simulink model "hqd_clarke"  (R2022b)
settings: Solver=FixedStepAuto  StartTime=0.0  StopTime=1.0  RelTol=1e-3
libraries: simulink x1
settings Model: Creator=15403  LastModifiedBy=15403
settings OptimizationCC: DefaultParameterBehavior=Inlined  UseDivisionForNetSlopeComputation=on  GainParamInheritBuiltInType=on  UseFloatMulNetSlope=on  InlineInvariantSignals=on  PassReuseOutputArgsAs=Individual arguments  ZeroExternalMemoryAtStartup=off  ZeroInternalMemoryAtStartup=off  NoFixptDivByZeroProtection=on  EfficientFloat2IntCast=on  LifeSpan=1  OptimizeBlockOrder=speed  DifferentSizesBufferReuse=on  EfficientTunableParamExpr=on
settings DebuggingCC: ParameterPrecisionLossMsg=none  ParameterTunabilityLossMsg=error
settings HardwareCC: ProdBitPerPointer=32  ProdBitPerSizeT=32  ProdBitPerPtrDiffT=32  ProdLargestAtomicInteger=Long  ProdLargestAtomicFloat=Double  ProdWordSize=32  ProdLongLongMode=on  ProdHWDeviceType=ARM Compatible->ARM Cortex-M
settings SFSimCC: MATLABDynamicMemAlloc=off
settings RTWCC: Description=Embedded Coder  SystemTargetFile=ert.tlc  TemplateMakefile=ert_default_tmf
settings CodeAppCC: ForceParamTrailComments=on  IgnoreCustomStorageClasses=off  OperatorAnnotations=on  SimulinkDataObjDesc=on  SFDataObjDesc=on  CustomSymbolStrGlobalVar=rt$N$M  CustomSymbolStrType=$N$M  CustomSymbolStrFcn=$N$M$F  CustomSymbolStrMacro=$N$M  InsertBlockDesc=on
settings ERTTargetCC: TargetLangStandard=C99 (ISO)  GenerateSampleERTMain=on  IncludeMdlTerminateFcn=off  CombineSignalStateStructs=on  SupportComplex=off  SupportContinuousTime=on  SupportNonInlinedSFcns=on  InlinedParameterPlacement=NonHierarchical  ERTCustomFileTemplate=example_file_process.tlc  ERTFilePackagingFormat=CompactWithDataFile

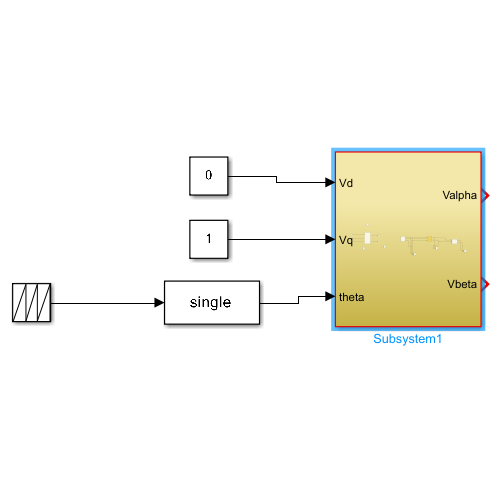
[thumbnail: Simulink's stored preview of the top-level diagram]
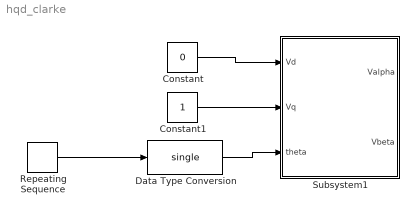
== system hqd_clarke ==
  Constant : Constant  Value=0  OutDataTypeStr=single
  Constant1 : Constant  OutDataTypeStr=single
  Data Type Conversion : DataTypeConversion  OutDataTypeStr=single  SaturateOnIntegerOverflow=off  RndMeth=Floor
  Repeating Sequence : simulink/Sources/Repeating Sequence  rep_seq_t=[0 0.1]  rep_seq_y=[0 2 * pi]
  Subsystem1 : Subsystem
  wires:
  Repeating Sequence/1 -> Data Type Conversion/1
  Constant/1 -> Subsystem1/1(Vd)
  Constant1/1 -> Subsystem1/2(Vq)
  Data Type Conversion/1 -> Subsystem1/3(theta)

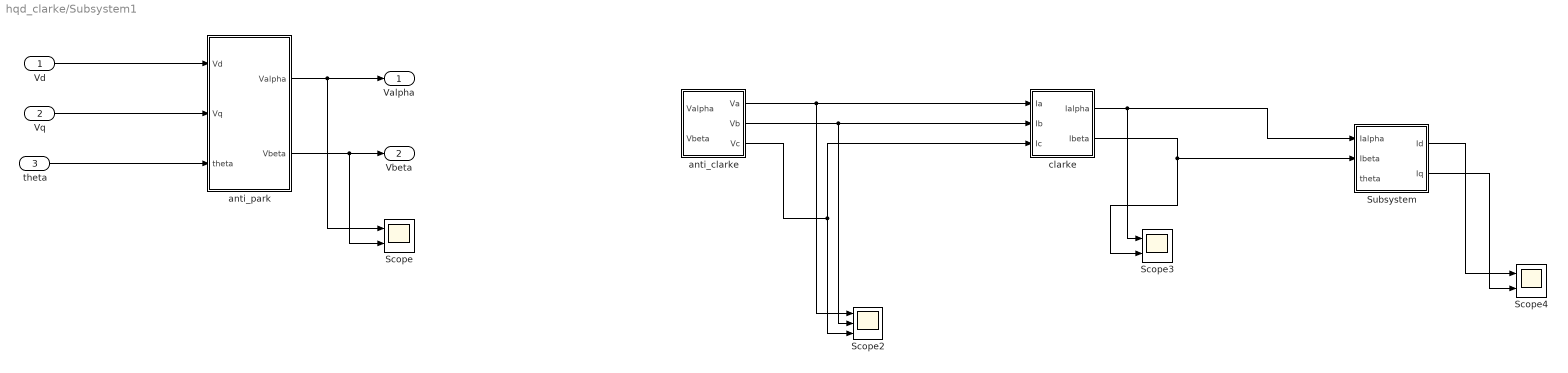
== system hqd_clarke/Subsystem1 ==
  Vd : Inport
  Vq : Inport  Port=2
  theta : Inport  Port=3
  Scope : Scope  NumInputPorts=2
  Scope2 : Scope  NumInputPorts=3
  Scope3 : Scope  NumInputPorts=2
  Scope4 : Scope  NumInputPorts=2
  Subsystem : Subsystem
  anti_clarke : Subsystem
  anti_park : Subsystem
  clarke : Subsystem
  Valpha : Outport
  Vbeta : Outport  Port=2
  wires:
  clarke/2(Ibeta) -> Scope3/2, Subsystem/2(Ibeta)
  anti_clarke/1(Va) -> clarke/1(Ia), Scope2/1
  Subsystem/1(Id) -> Scope4/1
  Subsystem/2(Iq) -> Scope4/2
  anti_clarke/3(Vc) -> clarke/3(Ic), Scope2/3
  anti_clarke/2(Vb) -> clarke/2(Ib), Scope2/2
  clarke/1(Ialpha) -> Subsystem/1(Ialpha), Scope3/1
  Vd/1 -> anti_park/1(Vd)
  Vq/1 -> anti_park/2(Vq)
  theta/1 -> anti_park/3(theta)
  anti_park/1(Valpha) -> Scope/1, Valpha/1
  anti_park/2(Vbeta) -> Scope/2, Vbeta/1

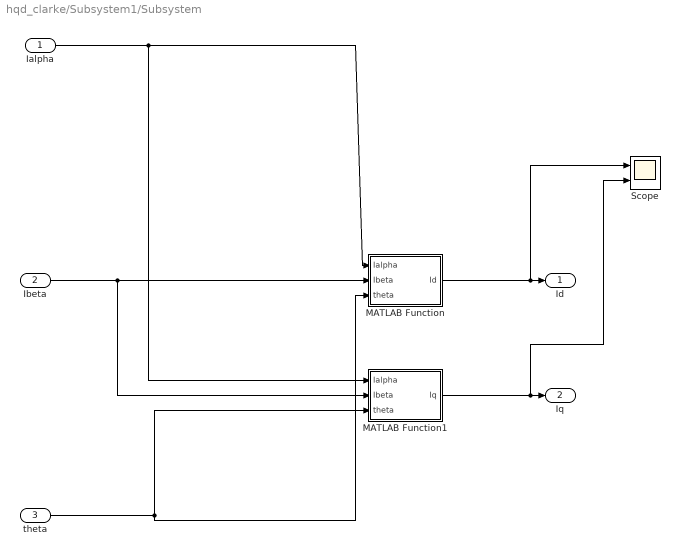
== system hqd_clarke/Subsystem1/Subsystem ==
  Ialpha : Inport
  Ibeta : Inport  Port=2
  theta : Inport  Port=3
  MATLAB Function : MATLAB Function  TreatAsAtomicUnit=on
  MATLAB Function1 : MATLAB Function  TreatAsAtomicUnit=on
  Scope : Scope  NumInputPorts=2
  Id : Outport
  Iq : Outport  Port=2
  wires:
  theta/1 -> MATLAB Function/3(theta), MATLAB Function1/3(theta)
  Ibeta/1 -> MATLAB Function/2(Ibeta), MATLAB Function1/2(Ibeta)
  MATLAB Function1/1(Iq) -> Scope/2, Iq/1
  MATLAB Function/1(Id) -> Scope/1, Id/1
  Ialpha/1 -> MATLAB Function/1(Ialpha), MATLAB Function1/1(Ialpha)

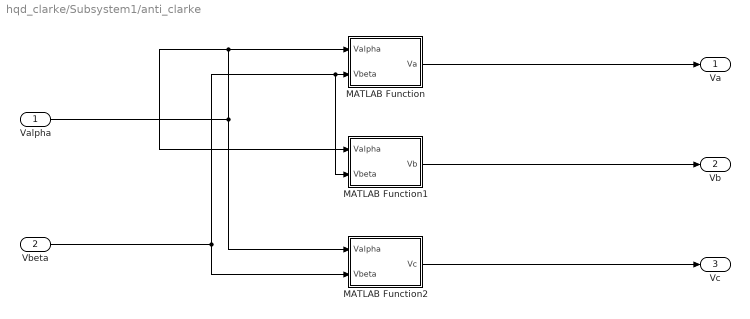
== system hqd_clarke/Subsystem1/anti_clarke ==
  " Valpha" : Inport
  Vbeta : Inport  Port=2
  MATLAB Function : MATLAB Function  TreatAsAtomicUnit=on
  MATLAB Function1 : MATLAB Function  TreatAsAtomicUnit=on
  MATLAB Function2 : MATLAB Function  TreatAsAtomicUnit=on
  Va : Outport
  Vb : Outport  Port=2
  Vc : Outport  Port=3
  wires:
  MATLAB Function/1(Va) -> Va/1
  Vbeta/1 -> MATLAB Function1/2(Vbeta), MATLAB Function/2(Vbeta), MATLAB Function2/2(Vbeta)
  " Valpha"/1 -> MATLAB Function/1(Valpha), MATLAB Function1/1(Valpha), MATLAB Function2/1(Valpha)
  MATLAB Function1/1(Vb) -> Vb/1
  MATLAB Function2/1(Vc) -> Vc/1

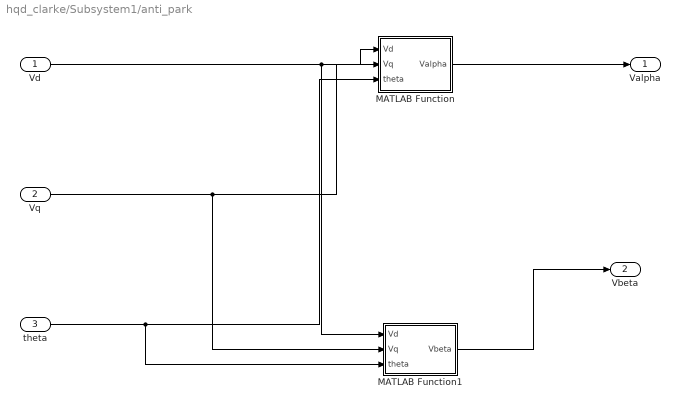
== system hqd_clarke/Subsystem1/anti_park ==
  Vd : Inport
  Vq : Inport  Port=2
  theta : Inport  Port=3
  MATLAB Function : MATLAB Function  TreatAsAtomicUnit=on
  MATLAB Function1 : MATLAB Function  TreatAsAtomicUnit=on
  Valpha : Outport
  Vbeta : Outport  Port=2
  wires:
  MATLAB Function/1(Valpha) -> Valpha/1
  MATLAB Function1/1(Vbeta) -> Vbeta/1
  Vd/1 -> MATLAB Function/1(Vd), MATLAB Function1/1(Vd)
  Vq/1 -> MATLAB Function/2(Vq), MATLAB Function1/2(Vq)
  theta/1 -> MATLAB Function/3(theta), MATLAB Function1/3(theta)

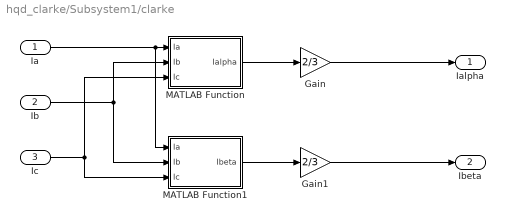
== system hqd_clarke/Subsystem1/clarke ==
  Ia : Inport
  Ib : Inport  Port=2
  Ic : Inport  Port=3
  Gain : Gain  Gain=2/3  OutDataTypeStr=single
  Gain1 : Gain  Gain=2/3  OutDataTypeStr=single
  MATLAB Function : MATLAB Function  TreatAsAtomicUnit=on
  MATLAB Function1 : MATLAB Function  TreatAsAtomicUnit=on
  Ialpha : Outport
  Ibeta : Outport  Port=2
  wires:
  Ia/1 -> MATLAB Function1/1(Ia), MATLAB Function/1(Ia)
  MATLAB Function/1(Ialpha) -> Gain/1
  Gain1/1 -> Ibeta/1
  Ib/1 -> MATLAB Function1/2(Ib), MATLAB Function/2(Ib)
  Ic/1 -> MATLAB Function/3(Ic), MATLAB Function1/3(Ic)
  MATLAB Function1/1(Ibeta) -> Gain1/1
  Gain/1 -> Ialpha/1

== matlab function hqd_clarke/Subsystem1/anti_park/MATLAB Function1 ==
  data: Vd input; Vbeta output; Vq input; theta input
function Vbeta = fcn(Vd, Vq, theta)

Vbeta = Vd * sin(theta) + Vq * cos(theta);

== matlab function hqd_clarke/Subsystem1/anti_park/MATLAB Function ==
  data: Vd input; Valpha output; Vq input; theta input
function Valpha = fcn(Vd, Vq, theta)

Valpha = Vd * cos(theta) - Vq * sin(theta);

== matlab function hqd_clarke/Subsystem1/anti_clarke/MATLAB Function ==
  data: Va output; Valpha input; Vbeta input
function Va = fcn(Valpha, Vbeta)

Va = Valpha;

== matlab function hqd_clarke/Subsystem1/anti_clarke/MATLAB Function1 ==
  data: Valpha input; Vb output; Vbeta input
function Vb = fcn(Valpha, Vbeta)

Vb = -Valpha * 1/2 + Vbeta * sqrt(3) / 2;

== matlab function hqd_clarke/Subsystem1/anti_clarke/MATLAB Function2 ==
  data: Valpha input; Vc output; Vbeta input
function Vc = fcn(Valpha, Vbeta)
Vc = -Valpha * 1/2 - Vbeta * sqrt(3) / 2;

== matlab function hqd_clarke/Subsystem1/clarke/MATLAB Function ==
  data: Ia input; Ialpha output; Ib input; Ic input
function Ialpha = fcn(Ia, Ib, Ic)

Ialpha = 3/2 * Ia;

== matlab function hqd_clarke/Subsystem1/clarke/MATLAB Function1 ==
  data: Ia input; Ibeta output; Ib input; Ic input
function Ibeta = fcn( Ia, Ib, Ic)

Ibeta = sqrt(3)/2 * (Ia + 2 * Ib);

== matlab function hqd_clarke/Subsystem1/Subsystem/MATLAB Function ==
  data: Ialpha input; Id output; Ibeta input; theta input
function Id = fcn(Ialpha, Ibeta, theta)

Id = Ialpha * cos(theta) + Ibeta * sin(theta);

== matlab function hqd_clarke/Subsystem1/Subsystem/MATLAB Function1 ==
  data: Ialpha input; Iq output; Ibeta input; theta input
function Iq = fcn(Ialpha, Ibeta, theta)
Iq = Ialpha * sin(theta) - Ibeta * cos(theta);
